simulink model "ids_android_app_stub"  (R2024a)
settings: Solver=FixedStepDiscrete  StartTime=0.0  StopTime=inf  FixedStep=0.1  RelTol=1e-3
settings Model: Creator=prana  LastModifiedBy=prana

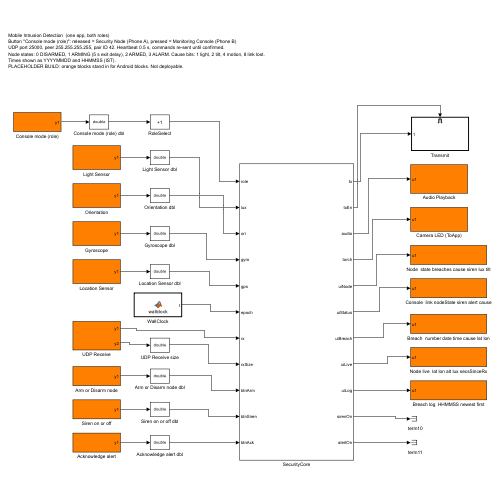
[thumbnail: Simulink's stored preview of the top-level diagram]
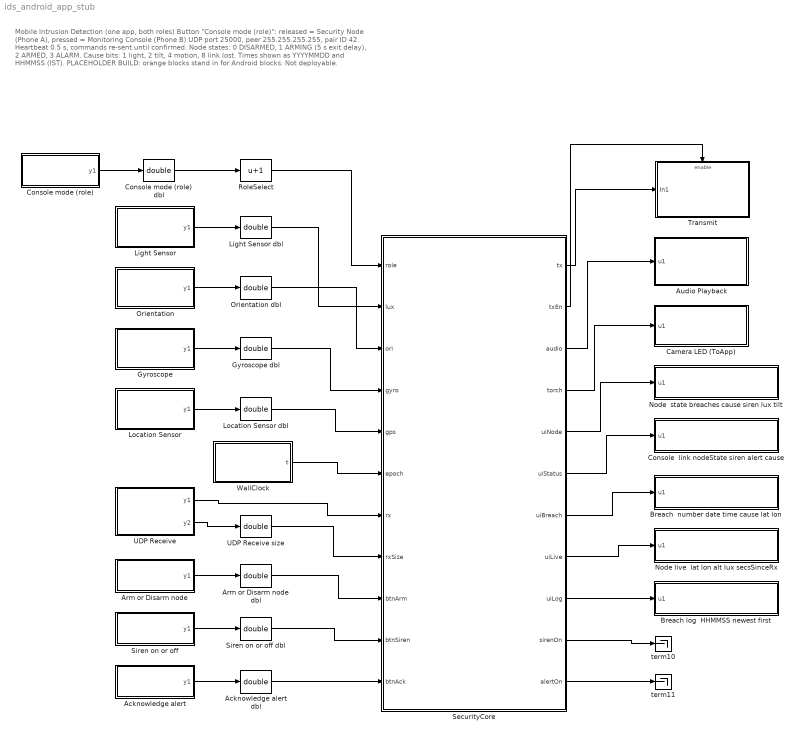
== system ids_android_app_stub ==
  note: Mobile Intrusion Detection  (one app, both roles)
      | Button "Console mode (role)": released = Security Node (Phone A), pressed = Monitoring Console (Phone B)
      | UDP port 25000, peer 255.255.255.255, pair ID 42. Heartbeat 0.5 s, commands re-sent until confirmed.
      | Node states: 0 DISARMED, 1 ARMING (5 s exit delay), 2 ARMED, 3 ALARM. Cause bits: 1 light, 2 tilt, 4 motion, 8 link lost.
      | Times shown as YYYYMMDD and HHMMSS (IST).
      | PLACEHOLDER BUILD: orange blocks stand in for Android blocks. Not deployable.
  Acknowledge alert : Subsystem
  Acknowledge alert dbl : DataTypeConversion  OutDataTypeStr=double  SaturateOnIntegerOverflow=off  RndMeth=Floor
  Arm or Disarm node : Subsystem
  Arm or Disarm node dbl : DataTypeConversion  OutDataTypeStr=double  SaturateOnIntegerOverflow=off  RndMeth=Floor
  Audio Playback : Subsystem
  Breach  number date time cause lat lon : Subsystem
  Breach log  HHMMSS newest first : Subsystem
  Camera LED (ToApp) : Subsystem
  Console  link nodeState siren alert cause : Subsystem
  Console mode (role) : Subsystem
  Console mode (role) dbl : DataTypeConversion  OutDataTypeStr=double  SaturateOnIntegerOverflow=off  RndMeth=Floor
  Gyroscope : Subsystem
  Gyroscope dbl : DataTypeConversion  OutDataTypeStr=double  SaturateOnIntegerOverflow=off  RndMeth=Floor
  Light Sensor : Subsystem
  Light Sensor dbl : DataTypeConversion  OutDataTypeStr=double  SaturateOnIntegerOverflow=off  RndMeth=Floor
  Location Sensor : Subsystem
  Location Sensor dbl : DataTypeConversion  OutDataTypeStr=double  SaturateOnIntegerOverflow=off  RndMeth=Floor
  Node  state breaches cause siren lux tilt : Subsystem
  Node live  lat lon alt lux secsSinceRx : Subsystem
  Orientation : Subsystem
  Orientation dbl : DataTypeConversion  OutDataTypeStr=double  SaturateOnIntegerOverflow=off  RndMeth=Floor
  RoleSelect : Bias  Bias=1  SaturateOnIntegerOverflow=off
  SecurityCore : Subsystem
  Siren on or off : Subsystem
  Siren on or off dbl : DataTypeConversion  OutDataTypeStr=double  SaturateOnIntegerOverflow=off  RndMeth=Floor
  Transmit : Subsystem  TreatAsAtomicUnit=on
  UDP Receive : Subsystem
  UDP Receive size : DataTypeConversion  OutDataTypeStr=double  SaturateOnIntegerOverflow=off  RndMeth=Floor
  WallClock : MATLAB Function  TreatAsAtomicUnit=on
  term10 : Terminator
  term11 : Terminator
  wires:
  UDP Receive/2(y2) -> UDP Receive size/1
  UDP Receive/1(y1) -> SecurityCore/7(rx)
  Console mode (role) dbl/1 -> RoleSelect/1
  UDP Receive size/1 -> SecurityCore/8(rxSize)
  Console mode (role)/1(y1) -> Console mode (role) dbl/1
  Light Sensor/1(y1) -> Light Sensor dbl/1
  Orientation dbl/1 -> SecurityCore/3(ori)
  Gyroscope/1(y1) -> Gyroscope dbl/1
  Gyroscope dbl/1 -> SecurityCore/4(gyro)
  Light Sensor dbl/1 -> SecurityCore/2(lux)
  Orientation/1(y1) -> Orientation dbl/1
  Location Sensor/1(y1) -> Location Sensor dbl/1
  Siren on or off dbl/1 -> SecurityCore/10(btnSiren)
  RoleSelect/1 -> SecurityCore/1(role)
  Arm or Disarm node/1(y1) -> Arm or Disarm node dbl/1
  Arm or Disarm node dbl/1 -> SecurityCore/9(btnArm)
  Siren on or off/1(y1) -> Siren on or off dbl/1
  SecurityCore/4(torch) -> Camera LED (ToApp)/1(u1)
  Acknowledge alert/1(y1) -> Acknowledge alert dbl/1
  Location Sensor dbl/1 -> SecurityCore/5(gps)
  WallClock/1(t) -> SecurityCore/6(epoch)
  SecurityCore/2(txEn) -> Transmit/Enable
  Acknowledge alert dbl/1 -> SecurityCore/11(btnAck)
  SecurityCore/5(uiNode) -> Node  state breaches cause siren lux tilt/1(u1)
  SecurityCore/1(tx) -> Transmit/1(In1)
  SecurityCore/3(audio) -> Audio Playback/1(u1)
  SecurityCore/10(sirenOn) -> term10/1
  SecurityCore/6(uiStatus) -> Console  link nodeState siren alert cause/1(u1)
  SecurityCore/11(alertOn) -> term11/1
  SecurityCore/7(uiBreach) -> Breach  number date time cause lat lon/1(u1)
  SecurityCore/8(uiLive) -> Node live  lat lon alt lux secsSinceRx/1(u1)
  SecurityCore/9(uiLog) -> Breach log  HHMMSS newest first/1(u1)

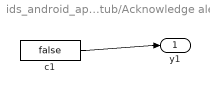
== system ids_android_app_stub/Acknowledge alert ==
  c1 : Constant  Value=false  SampleTime=0.1
  y1 : Outport
  wires:
  c1/1 -> y1/1

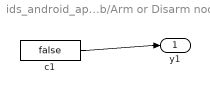
== system ids_android_app_stub/Arm or Disarm node ==
  c1 : Constant  Value=false  SampleTime=0.1
  y1 : Outport
  wires:
  c1/1 -> y1/1

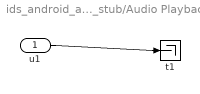
== system ids_android_app_stub/Audio Playback ==
  u1 : Inport
  t1 : Terminator
  wires:
  u1/1 -> t1/1

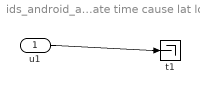
== system ids_android_app_stub/Breach  number date time cause lat lon ==
  u1 : Inport
  t1 : Terminator
  wires:
  u1/1 -> t1/1

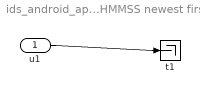
== system ids_android_app_stub/Breach log  HHMMSS newest first ==
  u1 : Inport
  t1 : Terminator
  wires:
  u1/1 -> t1/1

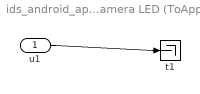
== system ids_android_app_stub/Camera LED (ToApp) ==
  u1 : Inport
  t1 : Terminator
  wires:
  u1/1 -> t1/1

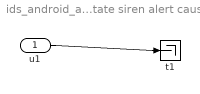
== system ids_android_app_stub/Console  link nodeState siren alert cause ==
  u1 : Inport
  t1 : Terminator
  wires:
  u1/1 -> t1/1

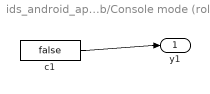
== system ids_android_app_stub/Console mode (role) ==
  c1 : Constant  Value=false  SampleTime=0.1
  y1 : Outport
  wires:
  c1/1 -> y1/1

== system ids_android_app_stub/Gyroscope ==
  c1 : Constant  Value=single([0 0 0])  SampleTime=0.1
  y1 : Outport
  wires:
  c1/1 -> y1/1

== system ids_android_app_stub/Light Sensor ==
  c1 : Constant  Value=single(0.5)  SampleTime=0.1
  y1 : Outport
  wires:
  c1/1 -> y1/1

== system ids_android_app_stub/Location Sensor ==
  c1 : Constant  Value=[0 0 0]  SampleTime=0.1
  y1 : Outport
  wires:
  c1/1 -> y1/1

== system ids_android_app_stub/Node  state breaches cause siren lux tilt ==
  u1 : Inport
  t1 : Terminator
  wires:
  u1/1 -> t1/1

== system ids_android_app_stub/Node live  lat lon alt lux secsSinceRx ==
  u1 : Inport
  t1 : Terminator
  wires:
  u1/1 -> t1/1

== system ids_android_app_stub/Orientation ==
  c1 : Constant  Value=single([0 0 0])  SampleTime=0.1
  y1 : Outport
  wires:
  c1/1 -> y1/1

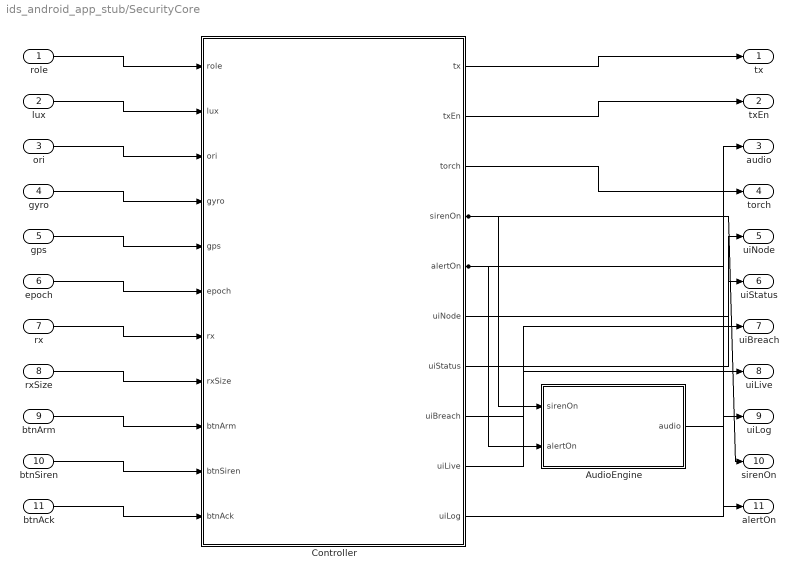
== system ids_android_app_stub/SecurityCore ==
  role : Inport
  lux : Inport  Port=2
  ori : Inport  Port=3
  gyro : Inport  Port=4
  gps : Inport  Port=5
  epoch : Inport  Port=6
  rx : Inport  Port=7
  rxSize : Inport  Port=8
  btnArm : Inport  Port=9
  btnSiren : Inport  Port=10
  btnAck : Inport  Port=11
  AudioEngine : MATLAB Function  TreatAsAtomicUnit=on
  Controller : MATLAB Function  TreatAsAtomicUnit=on
  tx : Outport
  txEn : Outport  Port=2
  audio : Outport  Port=3
  torch : Outport  Port=4
  uiNode : Outport  Port=5
  uiStatus : Outport  Port=6
  uiBreach : Outport  Port=7
  uiLive : Outport  Port=8
  uiLog : Outport  Port=9
  sirenOn : Outport  Port=10
  alertOn : Outport  Port=11
  wires:
  role/1 -> Controller/1(role)
  lux/1 -> Controller/2(lux)
  ori/1 -> Controller/3(ori)
  gyro/1 -> Controller/4(gyro)
  gps/1 -> Controller/5(gps)
  epoch/1 -> Controller/6(epoch)
  rx/1 -> Controller/7(rx)
  rxSize/1 -> Controller/8(rxSize)
  btnArm/1 -> Controller/9(btnArm)
  btnSiren/1 -> Controller/10(btnSiren)
  btnAck/1 -> Controller/11(btnAck)
  Controller/1(tx) -> tx/1
  Controller/2(txEn) -> txEn/1
  Controller/3(torch) -> torch/1
  Controller/4(sirenOn) -> AudioEngine/1(sirenOn), sirenOn/1
  Controller/5(alertOn) -> AudioEngine/2(alertOn), alertOn/1
  Controller/6(uiNode) -> uiNode/1
  Controller/7(uiStatus) -> uiStatus/1
  Controller/8(uiBreach) -> uiBreach/1
  Controller/9(uiLive) -> uiLive/1
  Controller/10(uiLog) -> uiLog/1
  AudioEngine/1(audio) -> audio/1

== system ids_android_app_stub/Siren on or off ==
  c1 : Constant  Value=false  SampleTime=0.1
  y1 : Outport
  wires:
  c1/1 -> y1/1

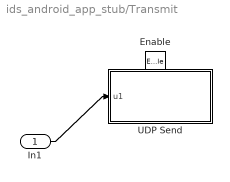
== system ids_android_app_stub/Transmit ==
  In1 : Inport
  Enable : EnablePort
  UDP Send : Subsystem
  wires:
  In1/1 -> UDP Send/1(u1)

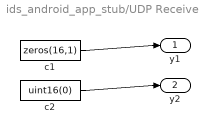
== system ids_android_app_stub/UDP Receive ==
  c1 : Constant  Value=zeros(16,1)  SampleTime=0.1
  c2 : Constant  Value=uint16(0)  SampleTime=0.1
  y1 : Outport
  y2 : Outport  Port=2
  wires:
  c1/1 -> y1/1
  c2/1 -> y2/1

== system ids_android_app_stub/Transmit/UDP Send ==
  u1 : Inport
  t1 : Terminator
  wires:
  u1/1 -> t1/1

== matlab function ids_android_app_stub/SecurityCore/AudioEngine ==
  data: sirenOn input; audio output; alertOn input
function audio = audio_engine(sirenOn, alertOn)
%#codegen
P = coder.const(ids_params());
persistent A
if isempty(A)
    A = audio_init();
end
S = coder.load('alert_message.mat', 'msg');
[A, audio] = audio_step(A, sirenOn, alertOn, S.msg, P);
end

== matlab function ids_android_app_stub/SecurityCore/Controller ==
  data: role input; tx output; lux input; ori input; gyro input; gps input; epoch input; rx input; rxSize input; btnArm input; btnSiren input; btnAck input; txEn output; torch output; sirenOn output; alertOn output; uiNode output; uiStatus output; uiBreach output; uiLive output; uiLog output
function [tx, txEn, torch, sirenOn, alertOn, uiNode, uiStatus, uiBreach, uiLive, uiLog] = controller(role, lux, ori, gyro, gps, epoch, rx, rxSize, btnArm, btnSiren, btnAck)
%#codegen
% Runs the Security Node and the Monitoring Console logic. Only the role
% selected by "role" is active, the other one is held in reset.
P = coder.const(ids_params());
persistent N C
if isempty(N)
    N = node_init();
    C = console_init(P.logLen);
end
isNode = double(role(1)) < 1.5;
rxd = double(rx(:));
rxs = double(rxSize(1));
t   = double(epoch(1));
[N, txN, enN, torchD, uiNode] = node_step(N, isNode, double(lux(1)), double(ori(:)'), double(gyro(:)'), double(gps(:)'), t, rxd, rxs, P);
[C, txC, enC, uiStatus, uiBreach, uiLive, uiLog] = console_step(C, ~isNode, double(btnArm(1)), double(btnSiren(1)), double(btnAck(1)), t, rxd, rxs, P);
if isNode
    tx = txN;
    txEn = enN;
else
    tx = txC;
    txEn = enC;
end
torch   = int32(torchD);
sirenOn = double(isNode && N.siren > 0);
alertOn = double(~isNode && C.alert > 0);
end

== matlab function ids_android_app_stub/WallClock ==
  settings: updateMethod=DISCRETE  sampleTime=0.1
  data: t output
function t = wallclock()
% Unix time from the phone clock (time(NULL) in the generated C)
t = wall_clock();
